simulink model "gantry_home_center_laser_servo"  (R2025b)
settings: Solver=FixedStepDiscrete  StartTime=0.0  StopTime=inf  FixedStep=0.05  RelTol=1e-3  EnableMultiTasking=on
libraries: raspberrypiBasiclib x6, simulink x2, raspberrypiNetworklib x1
settings Model: Creator=jeets  LastModifiedBy=jeets
settings SolverCC: PositivePriorityOrder=on
settings DataIOCC: ReturnWorkspaceOutputs=off
settings OptimizationCC: EnhancedBackFolding=on  PassReuseOutputArgsAs=Individual arguments  ZeroExternalMemoryAtStartup=off  ZeroInternalMemoryAtStartup=off  MaxStackSize=200000  OptimizeBlockOrder=speed  DifferentSizesBufferReuse=on  OptimizationCustomize=off  EfficientTunableParamExpr=on
settings DebuggingCC: ParameterTunabilityLossMsg=error
settings HardwareCC: ProdBitPerPointer=32.0  ProdBitPerSizeT=32.0  ProdBitPerPtrDiffT=32.0  ProdLargestAtomicInteger=Long  ProdLargestAtomicFloat=Double  ProdWordSize=32.0  ProdLongLongMode=on  ProdHWDeviceType=ARM Compatible->ARM Cortex-A (32-bit)
settings RTWCC: SystemTargetFile=ert.tlc  HardwareBoard=Raspberry Pi  TLCOptions="-aInlineSetEventsForThisBaseRateFcn=TLC_FALSE -aSuppressMultiTaskScheduler=TLC_FALSE  -aRateBasedStepFcn=0"  TemplateMakefile=ert_default_tmf  Toolchain=GNU GCC Embedded Linux  BuildConfiguration=Faster Runs  Description=Embedded Coder
settings CodeAppCC: ForceParamTrailComments=on  IgnoreCustomStorageClasses=off  OperatorAnnotations=on  SimulinkDataObjDesc=on  SFDataObjDesc=on  InsertBlockDesc=on
settings ERTTargetCC: ExtModeTransport=2.0  ExtModeStaticAlloc=on  ExtModeMexFile=ext_xcp  ExtModeIntrfLevel=Level2 - Open  InlinedParameterPlacement=Hierarchical  CodeReplacementLibrary=ARM Cortex-A CMSIS  SupportVariableSizeSignals=on

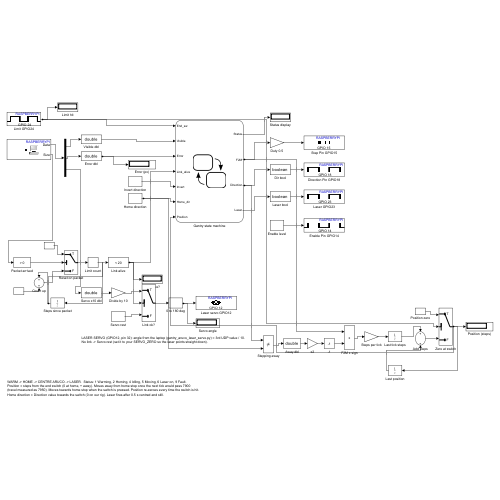
[thumbnail: Simulink's stored preview of the top-level diagram]
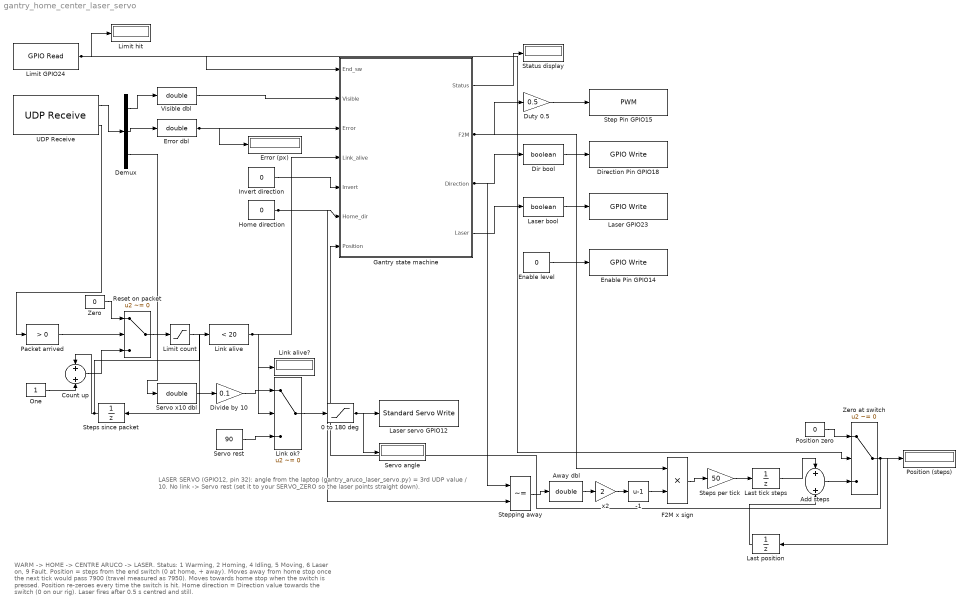
== system gantry_home_center_laser_servo ==
  note: WARM -> HOME -> CENTRE ARUCO -> LASER.  Status: 1 Warming, 2 Homing, 4 Idling, 5 Moving, 6 Laser on, 9 Fault.
      | Position = steps from the end switch (0 at home, + away). Moves away from home stop once the next tick would pass 7900
      | (travel measured as 7950). Moves towards home stop when the switch is pressed. Position re-zeroes every time the switch is hit.
      | Home direction = Direction value towards the switch (0 on our rig). Laser fires after 0.5 s centred and still.
  note: LASER SERVO (GPIO12, pin 32): angle from the laptop (gantry_aruco_laser_servo.py) = 3rd UDP value / 10.
      | No link -> Servo rest (set it to your SERVO_ZERO so the laser points straight down).
  -1 : Bias  Bias=-1  SaturateOnIntegerOverflow=off
  0 to 180 deg : Saturate  UpperLimit=180  LowerLimit=0
  Add steps : Sum
  Away dbl : DataTypeConversion  OutDataTypeStr=double  SaturateOnIntegerOverflow=off  RndMeth=Floor
  Count up : Sum
  Demux : Demux  Outputs=3
  Dir bool : DataTypeConversion  OutDataTypeStr=boolean  SaturateOnIntegerOverflow=off  RndMeth=Floor
  Direction Pin GPIO18 : raspberrypiBasiclib/GPIO Write  BoardProperty=Pi 3 Model B+  gpio=18  blockPlatform=Raspberry Pi  PinNumber=17  board=[]  direction=[]
  Divide by 10 : Gain  Gain=0.1
  Duty 0.5 : Gain  Gain=0.5
  Enable Pin GPIO14 : raspberrypiBasiclib/GPIO Write  BoardProperty=Pi 3 Model B+  gpio=14  blockPlatform=Raspberry Pi  PinNumber=17  board=[]  direction=[]
  Enable level : Constant  Value=0  OutDataTypeStr=boolean
  Error (px) : Display
  Error dbl : DataTypeConversion  OutDataTypeStr=double  SaturateOnIntegerOverflow=off  RndMeth=Floor
  F2M x sign : Product
  Gantry state machine : Stateflow chart  TreatAsAtomicUnit=on
  Home direction : Constant  Value=0
  Invert direction : Constant  Value=0
  Laser GPIO23 : raspberrypiBasiclib/GPIO Write  BoardProperty=Pi 3 Model B+  gpio=23  blockPlatform=Raspberry Pi  PinNumber=17  board=[]  direction=[]
  Laser bool : DataTypeConversion  OutDataTypeStr=boolean  SaturateOnIntegerOverflow=off  RndMeth=Floor
  Laser servo GPIO12 : raspberrypiBasiclib/Standard Servo Write  board=Pi 3 Model B+  Pin_=12  MinPulseDuration=1000e-6  MaxPulseDuration=2000e-6  blockPlatform=Raspberry Pi
  Last position : UnitDelay  SampleTime=0.05  HasFrameUpgradeWarning=on
  Last tick steps : UnitDelay  SampleTime=0.05  HasFrameUpgradeWarning=on
  Limit GPIO24 : raspberrypiBasiclib/GPIO Read  BoardProperty=Pi 3 Model B+  gpio=24  SampleTime=0.05  blockPlatform=Raspberry Pi  PinNumber=4  board=[]  direction=[]  internalResistor=[]
  Limit count : Saturate  UpperLimit=1000  LowerLimit=0
  Limit hit : Display
  Link alive : simulink/Logic and Bit Operations/Compare To Constant  relop=<  const=20  OutDataTypeStr=boolean
  Link alive? : Display
  Link ok? : Switch  Criteria=u2 ~= 0  SaturateOnIntegerOverflow=off  InputSameDT=off
  One : Constant
  Packet arrived : simulink/Logic and Bit Operations/Compare To Zero  relop=>  OutDataTypeStr=boolean
  Position (steps) : Display
  Position zero : Constant  Value=0
  Reset on packet : Switch  Criteria=u2 ~= 0  SaturateOnIntegerOverflow=off  InputSameDT=off
  Servo angle : Display
  Servo rest : Constant  Value=90
  Servo x10 dbl : DataTypeConversion  OutDataTypeStr=double  SaturateOnIntegerOverflow=off  RndMeth=Floor
  Status display : Display
  Step Pin GPIO15 : raspberrypiBasiclib/PWM  board=Pi 3 Model B+  Pin_=15  Frequency=1000  blockPlatform=Raspberry Pi
  Stepping away : RelationalOperator  Operator=~=  OutDataTypeStr=boolean  RndMeth=Simplest  InputSameDT=off
  Steps per tick : Gain  Gain=50
  Steps since packet : UnitDelay  InitialCondition=20  SampleTime=0.05  HasFrameUpgradeWarning=on
  UDP Receive : raspberrypiNetworklib/UDP Receive  localURL='0.0.0.0'  localPort=50001  remoteURL='0.0.0.0'  remotePort=-1  recvBufferSize=8192  signalDatatype=int16  dims=3  isVarSize=off  showBlockingTime=off  blockingTime=0  sampletime=0.05  blockPlatform=Raspberry Pi
  Visible dbl : DataTypeConversion  OutDataTypeStr=double  SaturateOnIntegerOverflow=off  RndMeth=Floor
  Zero : Constant  Value=0
  Zero at switch : Switch  Criteria=u2 ~= 0  SaturateOnIntegerOverflow=off  InputSameDT=off
  x2 : Gain  Gain=2
  wires:
  Limit GPIO24/1 -> Gantry state machine/1(End_sw), Limit hit/1, Zero at switch/2
  UDP Receive/1 -> Demux/1
  Demux/1 -> Visible dbl/1
  Visible dbl/1 -> Gantry state machine/2(Visible)
  Demux/2 -> Error dbl/1
  Error dbl/1 -> Gantry state machine/3(Error), Error (px)/1
  Link alive/1 -> Gantry state machine/4(Link_alive), Link alive?/1, Link ok?/2
  Invert direction/1 -> Gantry state machine/5(Invert)
  Home direction/1 -> Gantry state machine/6(Home_dir), Stepping away/2
  Zero at switch/1 -> Gantry state machine/7(Position), Last position/1, Position (steps)/1
  Gantry state machine/1(Status) -> Status display/1
  Gantry state machine/2(F2M) -> Duty 0.5/1, F2M x sign/1
  Duty 0.5/1 -> Step Pin GPIO15/1
  Gantry state machine/3(Direction) -> Dir bool/1, Stepping away/1
  Dir bool/1 -> Direction Pin GPIO18/1
  Gantry state machine/4(Laser) -> Laser bool/1
  Laser bool/1 -> Laser GPIO23/1
  Enable level/1 -> Enable Pin GPIO14/1
  UDP Receive/2 -> Packet arrived/1
  Zero/1 -> Reset on packet/1
  Packet arrived/1 -> Reset on packet/2
  Count up/1 -> Reset on packet/3
  Reset on packet/1 -> Limit count/1
  Limit count/1 -> Steps since packet/1
  Steps since packet/1 -> Count up/1, Link alive/1
  One/1 -> Count up/2
  Stepping away/1 -> Away dbl/1
  Away dbl/1 -> x2/1
  x2/1 -> -1/1
  -1/1 -> F2M x sign/2
  F2M x sign/1 -> Steps per tick/1
  Steps per tick/1 -> Last tick steps/1
  Last tick steps/1 -> Add steps/1
  Last position/1 -> Add steps/2
  Position zero/1 -> Zero at switch/1
  Add steps/1 -> Zero at switch/3
  Demux/3 -> Servo x10 dbl/1
  Servo x10 dbl/1 -> Divide by 10/1
  Divide by 10/1 -> Link ok?/1
  Servo rest/1 -> Link ok?/3
  Link ok?/1 -> 0 to 180 deg/1
  0 to 180 deg/1 -> Laser servo GPIO12/1, Servo angle/1

== stateflow chart gantry_home_center_laser_servo/Gantry state machine ==
  settings: updateMethod=DISCRETE  sampleTime=0.05
  state Warming
    en:
    Status = 1;
    F2M = 0;
    Laser = 0;
  state Homing
    en:
    Status = 2;
    Direction = Home_dir;
    F2M = 1;
  state Fault
    en:
    Status = 9;
    F2M = 0;
    Laser = 0;
  state Moving
    en, du:
    Status = 5;
    Direction = double(xor(Error > 0, Invert ~= 0));
    F2M = 1;
  state Idling
    en:
    Status = 4;
    F2M = 0;
    Laser = 0;
    Dwell = 0;
    du:
    if (Link_alive && Visible && abs(Error) < 40)
    Dwell = Dwell + 1;
    else
    Dwell = 0;
    end
  state Laser_On
    en:
    Status = 6;
    F2M = 0;
    Laser = 1;
  (default) -> Warming
  Warming -> Homing : after(5,sec)
  Homing -> Fault [order 2] : after(20,sec)
  Laser_On -> Idling : [~(Link_alive && Visible && abs(Error) < 40)]
  Idling -> Moving [order 1] : [Link_alive && Visible && abs(Error) > 40 && ~((End_sw == 1 && double(xor(Error > 0, Invert ~= 0)) == Home_dir) || (double(xor(Error > 0, Invert ~= 0)) ~= Home_dir && Position + 50 > 7900))]
  Homing -> Idling [order 1] : [End_sw == 1]
  Moving -> Idling : [~Link_alive || ~Visible || abs(Error) < 15 || ((End_sw == 1 && double(xor(Error > 0, Invert ~= 0)) == Home_dir) || (double(xor(Error > 0, Invert ~= 0)) ~= Home_dir && Position + 50 > 7900))]
  Idling -> Laser_On [order 2] : [Dwell >= 10]
  data: End_sw input; Visible input; Error input; Link_alive input; Invert input; Home_dir input; Position input; Status output double; F2M output double; Direction output double; Laser output double; Dwell local double =0
